simulink model "chaine_codee"  (R2023b)
settings: Solver=FixedStepDiscrete  StartTime=0.0  StopTime=Tsim  RelTol=1e-3
values from neighbouring files (symbols this model uses):
  A = P.A    [parametres.m]    (also in parametres_chaine.m; partie3_q4.m; partie3_q5.m; partie3_q8.m = 1)
  Ac = A * sqrt(R)    [partie4_q10.m]
  d_c = d    [partie4_q10.m]
  d_nc = d    [partie4_q10.m]
  dw = w    [partie4_q10.m]
  graine = 1    [extension_source_huffman.m]    (also in mes_parametres.m = mod(sum(c .* (1:numel(c)) * 31) + 7 * numel(c), 2^31 - 1); parametres_chaine.m = P.graine; parametres_perso.m = mod(sum(c .* (1:numel(c)) * 31) + 7 * numel(c), 2^31 - 1); partie4_q10.m = P.graine)
  L = cell(0, 2)    [construire_chaine_qpsk.m]    (also in construire_chaine_qpsk_codee.m; construire_chaine_texte.m; construire_decodeur_hamming.m = {'Mot recu/1', 'Bits r/1'; parametres.m = P.L)
  p1 = P.p1    [parametres.m]    (also in parametres_chaine.m = 0.5; partie3_q4.m; partie3_q5.m; partie3_q8.m = 0.3)
  seuil = 0    [parametres_chaine.m]    (also in partie4_q10.m)
  sigma2 = N0 * L / (2 * Tb)    [parametres_chaine.m]    (also in partie3_q12.m; partie4_q10.m)
  Tb = 1    [parametres.m]    (also in parametres_chaine.m; partie3_simulation.m; partie4_q10.m = 7; partie5_q2.m)
  Tc = R * Tb    (= 4)    [partie4_q10.m]
  Te_c = Tc / L    [partie4_q10.m]
  Te_nc = Tb / L    [partie4_q10.m]
libraries: simulink x7
settings Model: Creator=e2604176  LastModifiedBy=e2604176
settings OptimizationCC: BooleanDataType=off

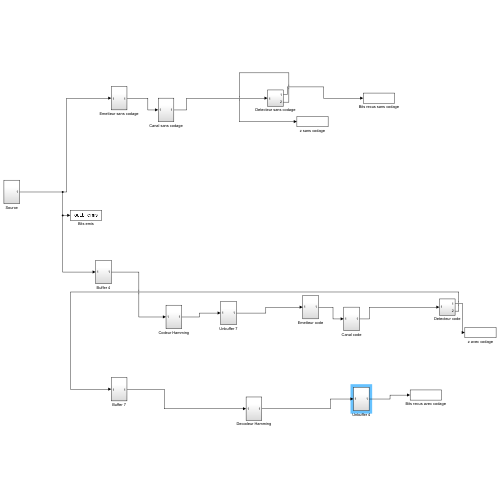
[thumbnail: Simulink's stored preview of the top-level diagram]
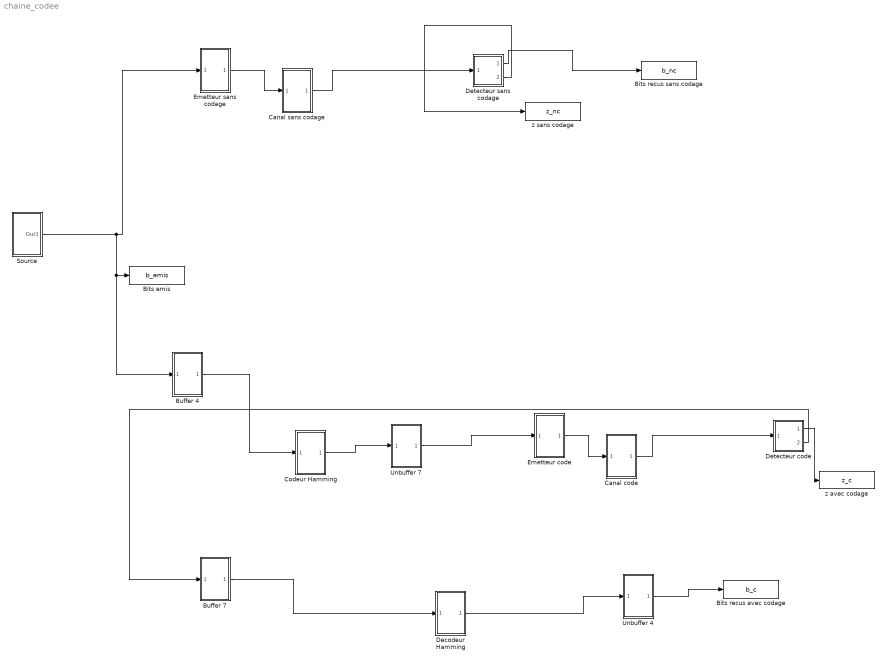
== system chaine_codee ==
  Bits emis : ToWorkspace  VariableName=b_emis  SampleTime=-1
  Bits recus avec codage : ToWorkspace  VariableName=b_c  SampleTime=-1
  Bits recus sans codage : ToWorkspace  VariableName=b_nc  SampleTime=-1
  Buffer 4 : Subsystem
  Buffer 7 : Subsystem
  Canal code : Subsystem
  Canal sans codage : Subsystem
  Codeur Hamming : Subsystem
  Decodeur Hamming : Subsystem
  Detecteur code : Subsystem
  Detecteur sans codage : Subsystem
  Emetteur code : Subsystem
  Emetteur sans codage : Subsystem
  Source : Subsystem
  Unbuffer 4 : Subsystem
  Unbuffer 7 : Subsystem
  z avec codage : ToWorkspace  VariableName=z_c  SampleTime=-1
  z sans codage : ToWorkspace  VariableName=z_nc  SampleTime=-1
  wires:
  Source/1(Out1) -> Emetteur sans codage/1(In1), Buffer 4/1(In1), Bits emis/1
  Emetteur sans codage/1(Out1) -> Canal sans codage/1(In1)
  Canal sans codage/1(Out1) -> Detecteur sans codage/1(In1)
  Detecteur sans codage/1(Out1) -> Bits recus sans codage/1
  Detecteur sans codage/2(Out2) -> z sans codage/1
  Buffer 4/1(Out1) -> Codeur Hamming/1(In1)
  Codeur Hamming/1(Out1) -> Unbuffer 7/1(In1)
  Unbuffer 7/1(Out1) -> Emetteur code/1(In1)
  Emetteur code/1(Out1) -> Canal code/1(In1)
  Canal code/1(Out1) -> Detecteur code/1(In1)
  Detecteur code/1(Out1) -> z avec codage/1
  Detecteur code/2(Out2) -> Buffer 7/1(In1)
  Buffer 7/1(Out1) -> Decodeur Hamming/1(In1)
  Decodeur Hamming/1(Out1) -> Unbuffer 4/1(In1)
  Unbuffer 4/1(Out1) -> Bits recus avec codage/1

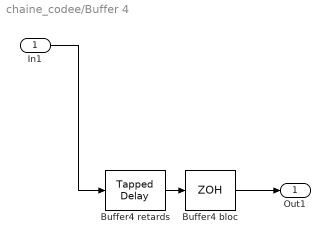
== system chaine_codee/Buffer 4 ==
  In1 : Inport
  Buffer4 bloc : ZeroOrderHold  SampleTime=4*Tb
  Buffer4 retards : simulink/Discrete/Tapped Delay  vinit=0  samptime=Tb  NumDelays=3  DelayOrder=Oldest  includeCurrent=on
  Out1 : Outport
  wires:
  Buffer4 retards/1 -> Buffer4 bloc/1
  In1/1 -> Buffer4 retards/1
  Buffer4 bloc/1 -> Out1/1

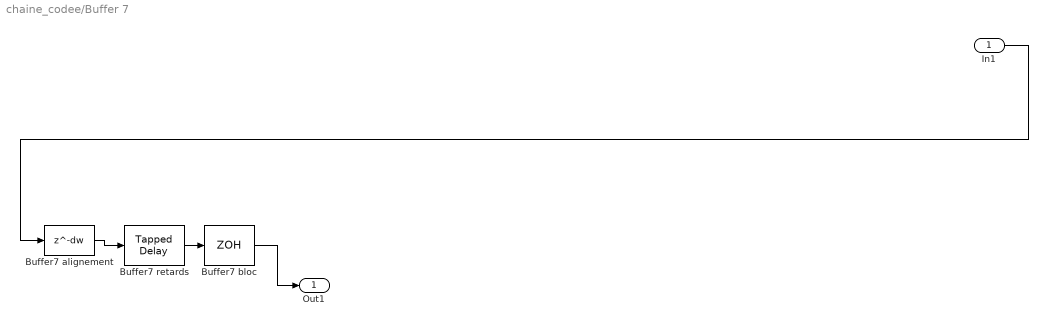
== system chaine_codee/Buffer 7 ==
  In1 : Inport
  Buffer7 alignement : Delay  DelayLength=dw
  Buffer7 bloc : ZeroOrderHold  SampleTime=4*Tb
  Buffer7 retards : simulink/Discrete/Tapped Delay  vinit=0  samptime=Tc  NumDelays=6  DelayOrder=Oldest  includeCurrent=on
  Out1 : Outport
  wires:
  Buffer7 alignement/1 -> Buffer7 retards/1
  In1/1 -> Buffer7 alignement/1
  Buffer7 retards/1 -> Buffer7 bloc/1
  Buffer7 bloc/1 -> Out1/1

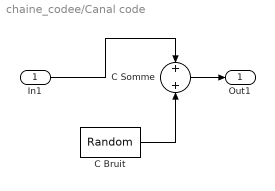
== system chaine_codee/Canal code ==
  In1 : Inport
  C Bruit : RandomNumber  Variance=sigma2  Seed=graine + 2  SampleTime=Te_c
  C Somme : Sum
  Out1 : Outport
  wires:
  C Bruit/1 -> C Somme/2
  In1/1 -> C Somme/1
  C Somme/1 -> Out1/1

== system chaine_codee/Canal sans codage ==
  In1 : Inport
  NC Bruit : RandomNumber  Variance=sigma2  Seed=graine + 1  SampleTime=Te_nc
  NC Somme : Sum
  Out1 : Outport
  wires:
  NC Somme/1 -> Out1/1
  NC Bruit/1 -> NC Somme/2
  In1/1 -> NC Somme/1

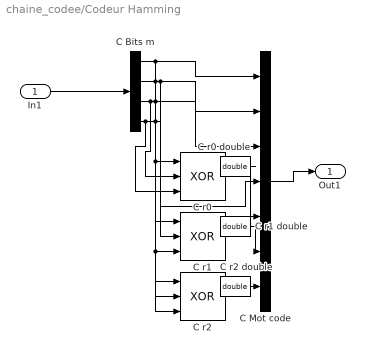
== system chaine_codee/Codeur Hamming ==
  In1 : Inport
  C Bits m : Demux
  C Mot code : Mux  Inputs=7
  C r0 : Logic  Operator=XOR  Inputs=3  AllPortsSameDT=off  OutDataTypeStr=boolean
  C r0 double : DataTypeConversion  OutDataTypeStr=double  SaturateOnIntegerOverflow=off  RndMeth=Floor
  C r1 : Logic  Operator=XOR  Inputs=3  AllPortsSameDT=off  OutDataTypeStr=boolean
  C r1 double : DataTypeConversion  OutDataTypeStr=double  SaturateOnIntegerOverflow=off  RndMeth=Floor
  C r2 : Logic  Operator=XOR  Inputs=3  AllPortsSameDT=off  OutDataTypeStr=boolean
  C r2 double : DataTypeConversion  OutDataTypeStr=double  SaturateOnIntegerOverflow=off  RndMeth=Floor
  Out1 : Outport
  wires:
  C Bits m/4 -> C r2/3, C Mot code/4, C r0/3
  C Bits m/1 -> C r0/1, C r1/1, C Mot code/1
  C Bits m/3 -> C r1/3, C r2/2, C Mot code/3, C r0/2
  C r0 double/1 -> C Mot code/5
  C Bits m/2 -> C r1/2, C Mot code/2, C r2/1
  C r1 double/1 -> C Mot code/6
  C r2/1 -> C r2 double/1
  C r2 double/1 -> C Mot code/7
  C r1/1 -> C r1 double/1
  C r0/1 -> C r0 double/1
  C Mot code/1 -> Out1/1
  In1/1 -> C Bits m/1

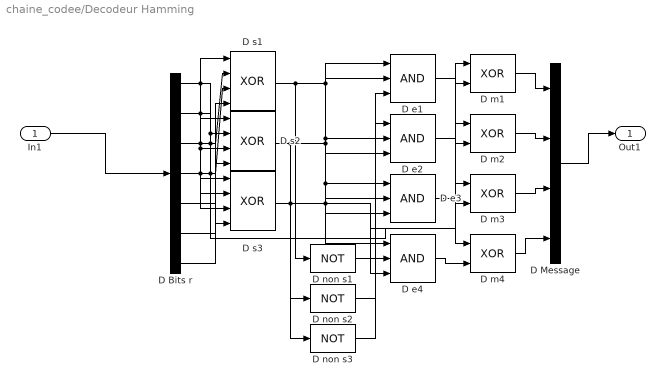
== system chaine_codee/Decodeur Hamming ==
  In1 : Inport
  D Bits r : Demux  Outputs=7
  D Message : Mux
  D e{1..4} (4 alike) : Logic  Inputs=3  AllPortsSameDT=off  OutDataTypeStr=boolean
  D m{1..4} (4 alike) : Logic  Operator=XOR  AllPortsSameDT=off  OutDataTypeStr=boolean
  D non s1 : Logic  Operator=NOT  Inputs=1  AllPortsSameDT=off  OutDataTypeStr=boolean
  D non s2 : Logic  Operator=NOT  Inputs=1  AllPortsSameDT=off  OutDataTypeStr=boolean
  D non s3 : Logic  Operator=NOT  Inputs=1  AllPortsSameDT=off  OutDataTypeStr=boolean
  D s1 : Logic  Operator=XOR  Inputs=4  AllPortsSameDT=off  OutDataTypeStr=boolean
  D s2 : Logic  Operator=XOR  Inputs=4  AllPortsSameDT=off  OutDataTypeStr=boolean
  D s3 : Logic  Operator=XOR  Inputs=4  AllPortsSameDT=off  OutDataTypeStr=boolean
  Out1 : Outport
  wires:
  D Bits r/2 -> D s2/2, D m2/1, D s3/1
  D Bits r/1 -> D s1/1, D s2/1, D m1/1
  D m1/1 -> D Message/1
  D s1/1 -> D e3/1, D e4/1, D e1/1, D non s1/1
  D non s1/1 -> D e2/1
  D s2/1 -> D e1/2, D e2/2, D e3/2, D non s2/1
  D m2/1 -> D Message/2
  D Bits r/4 -> D s1/3, D m4/1, D s3/3
  D Bits r/3 -> D s2/3, D s3/2, D s1/2, D m3/1
  D Bits r/5 -> D s1/4
  D Bits r/6 -> D s2/4
  D e3/1 -> D m3/2
  D s3/1 -> D e2/3, D e3/3, D e4/3, D non s3/1
  D e2/1 -> D m2/2
  D non s2/1 -> D e4/2
  D m3/1 -> D Message/3
  D e4/1 -> D m4/2
  D Message/1 -> Out1/1
  D m4/1 -> D Message/4
  D e1/1 -> D m1/2
  D non s3/1 -> D e1/3
  D Bits r/7 -> D s3/4
  In1/1 -> D Bits r/1

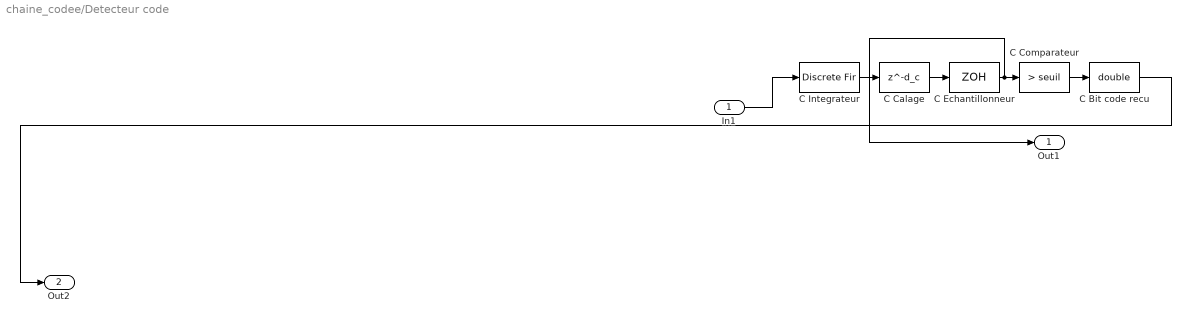
== system chaine_codee/Detecteur code ==
  In1 : Inport
  C Bit code recu : DataTypeConversion  OutDataTypeStr=double  SaturateOnIntegerOverflow=off  RndMeth=Floor
  C Calage : Delay  DelayLength=d_c
  C Comparateur : simulink/Logic and Bit Operations/Compare To Constant  relop=>  const=seuil  OutDataTypeStr=boolean
  C Echantillonneur : ZeroOrderHold  SampleTime=Tc
  C Integrateur : DiscreteFir  Coefficients=ones(1, L) / L  SampleTime=Te_c
  Out1 : Outport
  Out2 : Outport  Port=2
  wires:
  C Comparateur/1 -> C Bit code recu/1
  C Echantillonneur/1 -> Out1/1, C Comparateur/1
  C Integrateur/1 -> C Calage/1
  C Calage/1 -> C Echantillonneur/1
  In1/1 -> C Integrateur/1
  C Bit code recu/1 -> Out2/1

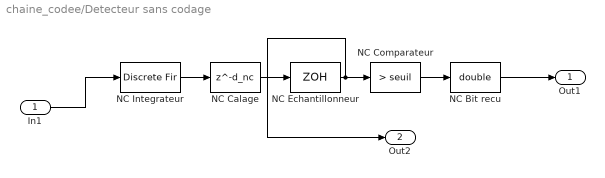
== system chaine_codee/Detecteur sans codage ==
  In1 : Inport
  NC Bit recu : DataTypeConversion  OutDataTypeStr=double  SaturateOnIntegerOverflow=off  RndMeth=Floor
  NC Calage : Delay  DelayLength=d_nc
  NC Comparateur : simulink/Logic and Bit Operations/Compare To Constant  relop=>  const=seuil  OutDataTypeStr=boolean
  NC Echantillonneur : ZeroOrderHold  SampleTime=Tb
  NC Integrateur : DiscreteFir  Coefficients=ones(1, L) / L  SampleTime=Te_nc
  Out1 : Outport
  Out2 : Outport  Port=2
  wires:
  NC Comparateur/1 -> NC Bit recu/1
  In1/1 -> NC Integrateur/1
  NC Echantillonneur/1 -> Out2/1, NC Comparateur/1
  NC Calage/1 -> NC Echantillonneur/1
  NC Integrateur/1 -> NC Calage/1
  NC Bit recu/1 -> Out1/1

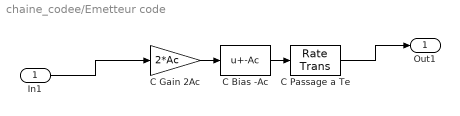
== system chaine_codee/Emetteur code ==
  In1 : Inport
  C Bias -Ac : Bias  Bias=-Ac  SaturateOnIntegerOverflow=off
  C Gain 2Ac : Gain  Gain=2*Ac
  C Passage a Te : RateTransition  OutPortSampleTime=Te_c
  Out1 : Outport
  wires:
  C Gain 2Ac/1 -> C Bias -Ac/1
  C Bias -Ac/1 -> C Passage a Te/1
  C Passage a Te/1 -> Out1/1
  In1/1 -> C Gain 2Ac/1

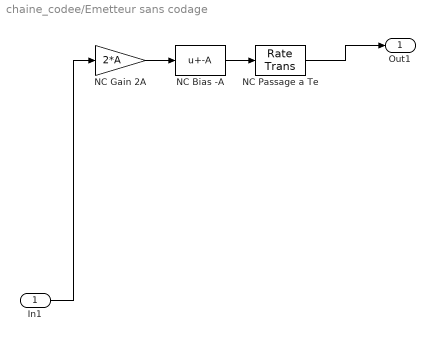
== system chaine_codee/Emetteur sans codage ==
  In1 : Inport
  NC Bias -A : Bias  Bias=-A  SaturateOnIntegerOverflow=off
  NC Gain 2A : Gain  Gain=2*A
  NC Passage a Te : RateTransition  OutPortSampleTime=Te_nc
  Out1 : Outport
  wires:
  NC Bias -A/1 -> NC Passage a Te/1
  NC Gain 2A/1 -> NC Bias -A/1
  In1/1 -> NC Gain 2A/1
  NC Passage a Te/1 -> Out1/1

== system chaine_codee/Source ==
  Bit : simulink/Logic and Bit Operations/Compare To Constant  relop=<  const=p1  OutDataTypeStr=boolean
  Bit double : DataTypeConversion  OutDataTypeStr=double  SaturateOnIntegerOverflow=off  RndMeth=Floor
  Uniforme : UniformRandomNumber  Minimum=0  Seed=graine  SampleTime=Tb
  Out1 : Outport
  wires:
  Bit/1 -> Bit double/1
  Uniforme/1 -> Bit/1
  Bit double/1 -> Out1/1

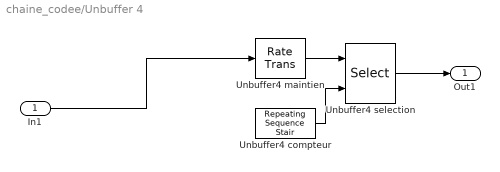
== system chaine_codee/Unbuffer 4 ==
  In1 : Inport
  Unbuffer4 compteur : simulink/Sources/Repeating Sequence Stair  OutValues=1:4  tsamp=Tb  OutMin=[]  OutMax=[]  OutDataTypeStr=double  OutputDataTypeScalingMode=double  OutDataType=fixdt(0,8)  ConRadixGroup=Best Precision: Vector-wise  OutScaling=2^-12
  Unbuffer4 maintien : RateTransition  OutPortSampleTime=Tb
  Unbuffer4 selection : Selector  InputPortWidth=4  IndexOptions=Index vector (port)  Indices=[1 3]  OutputSizes=1
  Out1 : Outport
  wires:
  Unbuffer4 maintien/1 -> Unbuffer4 selection/1
  Unbuffer4 compteur/1 -> Unbuffer4 selection/2
  Unbuffer4 selection/1 -> Out1/1
  In1/1 -> Unbuffer4 maintien/1

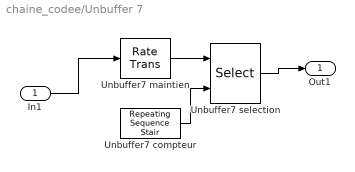
== system chaine_codee/Unbuffer 7 ==
  In1 : Inport
  Unbuffer7 compteur : simulink/Sources/Repeating Sequence Stair  OutValues=1:7  tsamp=Tc  OutMin=[]  OutMax=[]  OutDataTypeStr=double  OutputDataTypeScalingMode=double  OutDataType=fixdt(0,8)  ConRadixGroup=Best Precision: Vector-wise  OutScaling=2^-12
  Unbuffer7 maintien : RateTransition  OutPortSampleTime=Tc
  Unbuffer7 selection : Selector  InputPortWidth=7  IndexOptions=Index vector (port)  Indices=[1 3]  OutputSizes=1
  Out1 : Outport
  wires:
  In1/1 -> Unbuffer7 maintien/1
  Unbuffer7 compteur/1 -> Unbuffer7 selection/2
  Unbuffer7 maintien/1 -> Unbuffer7 selection/1
  Unbuffer7 selection/1 -> Out1/1
